simulink model "FOC"  (R2021a)
settings: Solver=VariableStepAuto  StartTime=0.0  StopTime=10  FixedStep=10e-5
InitFcn:
  | cd 'F:\Learning\Power\FOC';
  | run('Params.m')
values from neighbouring files (symbols this model uses):
  B = 1e-4    (= 0.0001)    [Params.m]
  Id_max = -62.5    [Params.m]
  Iq_max = 62.5    [Params.m]
  Is_max = 125    [Params.m]
  J = 0.004    [Params.m]
  Ka_id = 1 / Kp_id    (= 0.0111111111111)    [Params.m]
  Ka_iq = 1 / Kp_iq    (= 2.06143063286)    [Params.m]
  Ka_w = 1 / Kp_w    (= 0.1)    [Params.m]
  Kest = Rs/Ls    (= 212.401995723)    [Params.m]
  Ki_id = 50    [Params.m]
  Ki_iq = 93.62    [Params.m]
  Ki_w = 15    [Params.m]
  Kp_id = 90    [Params.m]
  Kp_iq = 0.4851    [Params.m]
  Kp_ll = 2500000    [Params.m]
  Kp_w = 10    [Params.m]
  Kw_Y = 7.98e-3    (= 0.00798)    [Params.m]
  Ld = 6.31e-5    (= 6.31e-05)    [Params.m]
  Lq = 7.72e-5    (= 7.72e-05)    [Params.m]
  Ls = 7.015e-5    (= 7.015e-05)    [Params.m]
  p = 6    [Params.m]
  Rs = 0.0149    [Params.m]
  Te_max = 2.4    [Params.m]
  Te_min = -2.4    [Params.m]
  TL = 1.67    [Params.m]
  Ts = 1/fs    (= 5e-05)    [Params.m]
  Vs_max = V_DC / sqrt(3)    [Params.m]
  Ypm = 7.89e-3    (= 0.00789)    [Params.m]
undefined symbols (not defined in the file or in its folder): magnitude
libraries: spsMosfetLib x6, spsVoltageMeasurementLib x3, spsDCVoltageSourceLib x2, spsGroundLib x1, spspowerguiLib x1
settings Model: SimulationMode=rapid-accelerator  Creator=DEEL  LastModifiedBy=DEEL
settings SolverCC: ZeroCrossControl=DisableAll
settings OptimizationCC: DefaultParameterBehavior=Inlined  EnhancedBackFolding=on  PassReuseOutputArgsAs=Individual arguments  ZeroExternalMemoryAtStartup=off  ZeroInternalMemoryAtStartup=off  OptimizeBlockOrder=speed  DifferentSizesBufferReuse=on  OptimizationCustomize=off  EfficientTunableParamExpr=on
settings DebuggingCC: ParameterTunabilityLossMsg=error
settings SFSimCC: MATLABDynamicMemAlloc=off
settings RTWCC: SystemTargetFile=ert.tlc  TemplateMakefile=ert_default_tmf
settings CodeAppCC: ForceParamTrailComments=on  IgnoreCustomStorageClasses=off  OperatorAnnotations=on  SimulinkDataObjDesc=on  SFDataObjDesc=on  InsertBlockDesc=on
settings ERTTargetCC: TargetLangStandard=C99 (ISO)  GenerateSampleERTMain=on  InlinedParameterPlacement=NonHierarchical  RTWCAPISignals=on  RTWCAPIParams=on  ERTCustomFileTemplate=example_file_process.tlc

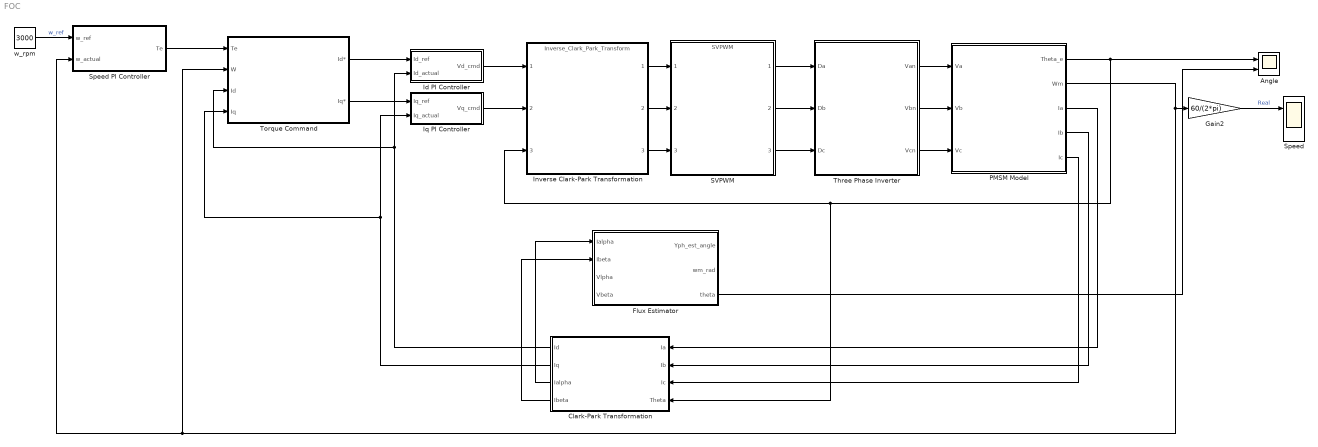
== system FOC ==
  Angle : Scope  NumInputPorts=2
  Clark-Park Transformation : Subsystem
  Flux Estimator : Subsystem
  Gain2 : Gain  Gain=60/(2*pi)
  Id PI Controller : Subsystem
  Inverse Clark-Park Transformation : ModelReference  ModelNameDialog=Inverse_Clark_Park_Transform  SimulationMode=Normal  ModelReferenceVersion=1.215
  Iq PI Controller : Subsystem
  PMSM Model : Subsystem
  SVPWM : ModelReference  ModelNameDialog=SVPWM  SimulationMode=Normal  ModelReferenceVersion=1.224
  Speed : Scope  NumInputPorts=2
  Speed PI Controller : Subsystem
  Three Phase Inverter : Subsystem
  Torque Command : Subsystem
  w_rpm : Constant  Value=3000
  wires:
  w_rpm/1 -> Speed PI Controller/1(w_ref)  "w_ref"
  Speed PI Controller/1(Te) -> Torque Command/1(Te)
  Id PI Controller/1(Vd_cmd) -> Inverse Clark-Park Transformation/1
  Iq PI Controller/1(Vq_cmd) -> Inverse Clark-Park Transformation/2
  Torque Command/1(Id*) -> Id PI Controller/1(Id_ref)
  SVPWM/3 -> Three Phase Inverter/3(Dc)
  SVPWM/1 -> Three Phase Inverter/1(Da)
  Inverse Clark-Park Transformation/1 -> SVPWM/1
  Inverse Clark-Park Transformation/2 -> SVPWM/2
  Inverse Clark-Park Transformation/3 -> SVPWM/3
  Clark-Park Transformation/1(Id) -> Torque Command/3(Id), Id PI Controller/2(Id_actual)
  Three Phase Inverter/1(Van) -> PMSM Model/1(Va)
  Three Phase Inverter/3(Vcn) -> PMSM Model/3(Vc)
  PMSM Model/3(Ia) -> Clark-Park Transformation/1(Ia)
  PMSM Model/4(Ib) -> Clark-Park Transformation/2(Ib)
  PMSM Model/5(Ic) -> Clark-Park Transformation/3(Ic)
  PMSM Model/2(Wm) -> Torque Command/2(W), Speed PI Controller/2(w_actual), Gain2/1
  PMSM Model/1(Theta_e) -> Clark-Park Transformation/4(Theta), Inverse Clark-Park Transformation/3, Angle/1
  Clark-Park Transformation/2(Iq) -> Torque Command/4(Iq), Iq PI Controller/2(Iq_actual)
  Three Phase Inverter/2(Vbn) -> PMSM Model/2(Vb)
  SVPWM/2 -> Three Phase Inverter/2(Db)
  Gain2/1 -> Speed/1  "Real"
  Torque Command/2(Iq*) -> Iq PI Controller/1(Iq_ref)
  Clark-Park Transformation/3(Ialpha) -> Flux Estimator/1(Ialpha)
  Clark-Park Transformation/4(Ibeta) -> Flux Estimator/2(Ibeta)
  Flux Estimator/3(theta) -> Angle/2

== system FOC/Clark-Park Transformation ==
  Ia : Inport
  Ib : Inport  Port=2
  Ic : Inport  Port=3
  Theta : Inport  Port=4
  Clark Transformation : Subsystem
  Park Transformation : Subsystem
  Id : Outport
  Iq : Outport  Port=2
  Ialpha : Outport  Port=3
  Ibeta : Outport  Port=4
  wires:
  Theta/1 -> Park Transformation/3(Theta)
  Clark Transformation/2(Vbeta) -> Ibeta/1, Park Transformation/2(Vbeta)
  Clark Transformation/1(Valpha) -> Ialpha/1, Park Transformation/1(Valpha)
  Ic/1 -> Clark Transformation/3(Vc)
  Ib/1 -> Clark Transformation/2(Vb)
  Ia/1 -> Clark Transformation/1(Va)
  Park Transformation/2(Vq) -> Iq/1
  Park Transformation/1(Vd) -> Id/1

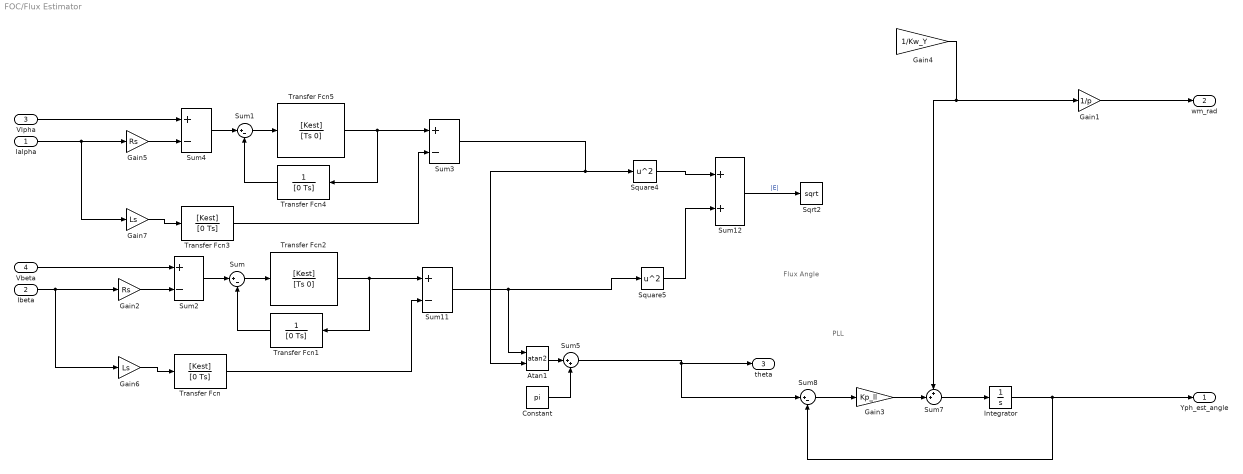
== system FOC/Flux Estimator ==
  note: PLL
  note: Flux Angle
  Ialpha : Inport
  Ibeta : Inport  Port=2
  Vlpha : Inport  Port=3
  Vbeta : Inport  Port=4
  Atan1 : Trigonometry  Operator=atan2
  Constant : Constant  Value=pi
  Gain1 : Gain  Gain=1/p
  Gain2 : Gain  Gain=Rs
  Gain3 : Gain  Gain=Kp_ll
  Gain4 : Gain  Gain=1/Kw_Y
  Gain5 : Gain  Gain=Rs
  Gain6 : Gain  Gain=Ls
  Gain7 : Gain  Gain=Ls
  Integrator : Integrator
  Sqrt2 : Sqrt  SaturateOnIntegerOverflow=on
  Square4 : Math  Operator=square  SaturateOnIntegerOverflow=on
  Square5 : Math  Operator=square  SaturateOnIntegerOverflow=on
  Sum : Sum  Inputs=|+-
  Sum1 : Sum  Inputs=|+-
  Sum{2..4,11} (4 alike) : Sum  Inputs=+-
  Sum12 : Sum
  Sum5 : Sum  Inputs=|++
  Sum7 : Sum  Inputs=++|
  Sum8 : Sum  Inputs=|+-
  Transfer Fcn : TransferFcn  Numerator=[Kest]  Denominator=[0 Ts]
  Transfer Fcn1 : TransferFcn  Denominator=[0 Ts]
  Transfer Fcn2 : TransferFcn  Numerator=[Kest]  Denominator=[Ts 0]
  Transfer Fcn3 : TransferFcn  Numerator=[Kest]  Denominator=[0 Ts]
  Transfer Fcn4 : TransferFcn  Denominator=[0 Ts]
  Transfer Fcn5 : TransferFcn  Numerator=[Kest]  Denominator=[Ts 0]
  Yph_est_angle : Outport
  wm_rad : Outport  Port=2
  theta : Outport  Port=3
  wires:
  Gain2/1 -> Sum2/2
  Ibeta/1 -> Gain6/1, Gain2/1
  Gain1/1 -> wm_rad/1
  Sum7/1 -> Integrator/1
  Sum8/1 -> Gain3/1
  Vbeta/1 -> Sum2/1
  Gain4/1 -> Sum7/1, Gain1/1
  Integrator/1 -> Yph_est_angle/1, Sum8/2
  Gain3/1 -> Sum7/2
  Square5/1 -> Sum12/2
  Square4/1 -> Sum12/1
  Sum12/1 -> Sqrt2/1  "|E|"
  Sum3/1 -> Atan1/2, Square4/1
  Sum11/1 -> Square5/1, Atan1/1
  Sum5/1 -> Sum8/1, theta/1
  Gain6/1 -> Transfer Fcn/1
  Sum/1 -> Transfer Fcn2/1
  Sum2/1 -> Sum/1
  Transfer Fcn1/1 -> Sum/2
  Transfer Fcn2/1 -> Transfer Fcn1/1, Sum11/1
  Transfer Fcn/1 -> Sum11/2
  Transfer Fcn3/1 -> Sum3/2
  Transfer Fcn5/1 -> Sum3/1, Transfer Fcn4/1
  Transfer Fcn4/1 -> Sum1/2
  Sum4/1 -> Sum1/1
  Sum1/1 -> Transfer Fcn5/1
  Gain7/1 -> Transfer Fcn3/1
  Vlpha/1 -> Sum4/1
  Ialpha/1 -> Gain7/1, Gain5/1
  Gain5/1 -> Sum4/2
  Atan1/1 -> Sum5/1
  Constant/1 -> Sum5/2

== system FOC/Id PI Controller ==
  Id_ref : Inport
  Id_actual : Inport  Port=2
  Gain : Gain  Gain=Kp_id
  Gain1 : Gain  Gain=Ki_id
  Gain2 : Gain  Gain=Ka_id
  Integrator : Integrator
  Saturation : Saturate  UpperLimit=Vs_max  LowerLimit=-Vs_max
  Sum : Sum  Inputs=|+-
  Sum1 : Sum  Inputs=|++
  Sum2 : Sum  Inputs=+-|
  Sum3 : Sum  Inputs=|+-
  Vd_cmd : Outport
  wires:
  Sum1/1 -> Sum2/1, Saturation/1  "Voltage_Command"
  Integrator/1 -> Sum1/2
  Gain/1 -> Sum1/1
  Gain1/1 -> Integrator/1
  Sum/1 -> Sum3/1, Gain/1  "Id_err"
  Id_actual/1 -> Sum/2
  Id_ref/1 -> Sum/1
  Sum2/1 -> Gain2/1
  Gain2/1 -> Sum3/2  "Anti-WindUp"
  Saturation/1 -> Sum2/2, Vd_cmd/1
  Sum3/1 -> Gain1/1  "Id_err"

== system FOC/Iq PI Controller ==
  Iq_ref : Inport
  Iq_actual : Inport  Port=2
  Gain : Gain  Gain=Kp_iq
  Gain1 : Gain  Gain=Ki_iq
  Gain2 : Gain  Gain=Ka_iq
  Integrator : Integrator
  Saturation1 : Saturate  UpperLimit=Vs_max  LowerLimit=-Vs_max
  Sum : Sum  Inputs=|+-
  Sum1 : Sum  Inputs=|++
  Sum2 : Sum  Inputs=+-|
  Sum3 : Sum  Inputs=|+-
  Vq_cmd : Outport
  wires:
  Gain1/1 -> Integrator/1
  Gain/1 -> Sum1/1
  Integrator/1 -> Sum1/2
  Sum1/1 -> Sum2/1, Saturation1/1  "Voltage_Command"
  Iq_actual/1 -> Sum/2
  Iq_ref/1 -> Sum/1
  Sum2/1 -> Gain2/1
  Saturation1/1 -> Sum2/2, Vq_cmd/1
  Gain2/1 -> Sum3/2  "Anti-WindUp"
  Sum/1 -> Sum3/1, Gain/1  "Iq_err"
  Sum3/1 -> Gain1/1  "Iq_err"

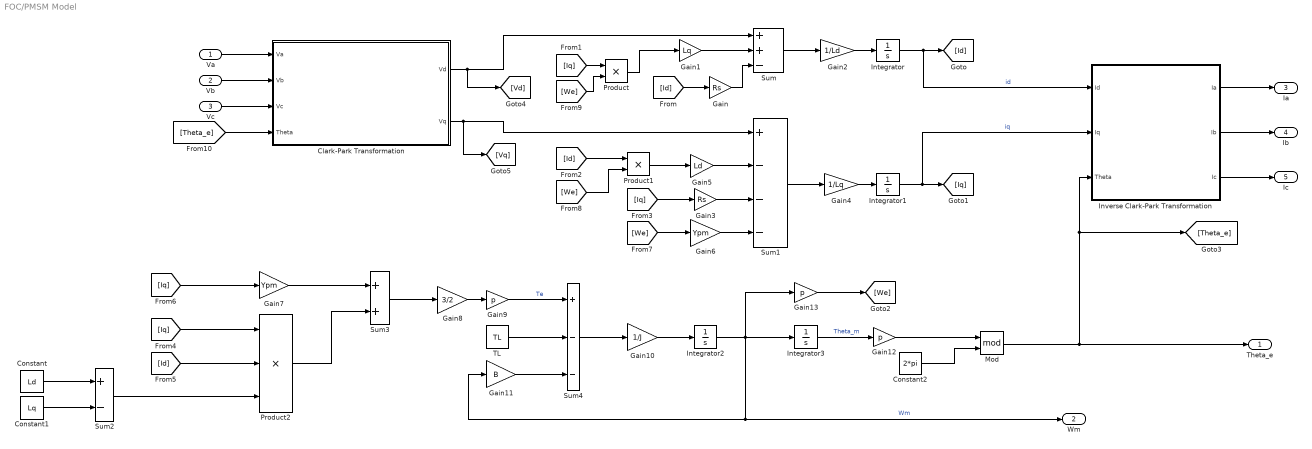
== system FOC/PMSM Model ==
  Va : Inport
  Vb : Inport  Port=2
  Vc : Inport  Port=3
  Clark-Park Transformation : Subsystem
  Constant : Constant  Value=Ld
  Constant1 : Constant  Value=Lq
  Constant2 : Constant  Value=2*pi
  Gain : Gain  Gain=Rs
  Gain1 : Gain  Gain=Lq
  Gain10 : Gain  Gain=1/J
  Gain11 : Gain  Gain=B
  Gain12 : Gain  Gain=p
  Gain13 : Gain  Gain=p
  Gain2 : Gain  Gain=1/Ld
  Gain3 : Gain  Gain=Rs
  Gain4 : Gain  Gain=1/Lq
  Gain5 : Gain  Gain=Ld
  Gain6 : Gain  Gain=Ypm
  Gain7 : Gain  Gain=Ypm
  Gain8 : Gain  Gain=3/2
  Gain9 : Gain  Gain=p
  Integrator{,1..3} (4 alike) : Integrator
  Inverse Clark-Park Transformation : Subsystem
  Mod : Math  Operator=mod  SaturateOnIntegerOverflow=on
  Product : Product
  Product1 : Product
  Product2 : Product  Inputs=3
  Sum : Sum  Inputs=++-
  Sum1 : Sum  Inputs=+---
  Sum2 : Sum  Inputs=+-
  Sum3 : Sum
  Sum4 : Sum  Inputs=+--
  TL : Constant  Value=TL
  Theta_e : Outport
  Wm : Outport  Port=2
  Ia : Outport  Port=3
  Ib : Outport  Port=4
  Ic : Outport  Port=5
  wires:
  Vc/1 -> Clark-Park Transformation/3(Vc)
  Va/1 -> Clark-Park Transformation/1(Va)
  Clark-Park Transformation/1(Vd) -> [Vd], Sum/1
  Gain/1 -> Sum/3
  Product/1 -> Gain1/1
  Sum/1 -> Gain2/1
  Gain2/1 -> Integrator/1
  Gain1/1 -> Sum/2
  Clark-Park Transformation/2(Vq) -> [Vq], Sum1/1
  Sum1/1 -> Gain4/1
  Gain4/1 -> Integrator1/1
  Gain3/1 -> Sum1/3
  Product1/1 -> Gain5/1
  Gain5/1 -> Sum1/2
  Integrator/1 -> Inverse Clark-Park Transformation/1(Id), [Id]  "id"
  [Id] -> Gain/1
  Integrator1/1 -> Inverse Clark-Park Transformation/2(Iq), [Iq]  "iq"
  [Iq] -> Product/1
  [Id] -> Product1/1
  [Iq] -> Gain3/1
  Gain6/1 -> Sum1/4
  [Iq] -> Product2/1
  [Id] -> Product2/2
  Sum2/1 -> Product2/3
  Constant1/1 -> Sum2/2
  Constant/1 -> Sum2/1
  [Iq] -> Gain7/1
  Gain7/1 -> Sum3/1
  Product2/1 -> Sum3/2
  Sum3/1 -> Gain8/1
  Sum4/1 -> Gain10/1
  TL/1 -> Sum4/2
  Gain11/1 -> Sum4/3
  Gain10/1 -> Integrator2/1
  Integrator2/1 -> Gain13/1, Integrator3/1, Wm/1, Gain11/1  "Wm"
  Integrator3/1 -> Gain12/1  "Theta_m"
  Gain13/1 -> [We]
  [We] -> Gain6/1
  [We] -> Product1/2
  [We] -> Product/2
  Gain12/1 -> Mod/1
  Constant2/1 -> Mod/2
  [Theta_e] -> Clark-Park Transformation/4(Theta)
  Gain8/1 -> Gain9/1
  Gain9/1 -> Sum4/1  "Te"
  Mod/1 -> Theta_e/1, Inverse Clark-Park Transformation/3(Theta), [Theta_e]
  Vb/1 -> Clark-Park Transformation/2(Vb)
  Inverse Clark-Park Transformation/1(Ia) -> Ia/1
  Inverse Clark-Park Transformation/2(Ib) -> Ib/1
  Inverse Clark-Park Transformation/3(Ic) -> Ic/1

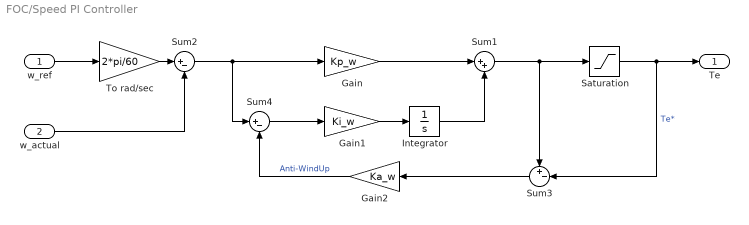
== system FOC/Speed PI Controller ==
  w_ref : Inport
  w_actual : Inport  Port=2
  Gain : Gain  Gain=Kp_w
  Gain1 : Gain  Gain=Ki_w
  Gain2 : Gain  Gain=Ka_w
  Integrator : Integrator
  Saturation : Saturate  UpperLimit=Te_max  LowerLimit=Te_min
  Sum1 : Sum  Inputs=|++
  Sum2 : Sum  Inputs=|+-
  Sum3 : Sum  Inputs=+-|
  Sum4 : Sum  Inputs=|+-
  To rad/sec : Gain  Gain=2*pi/60
  Te : Outport
  wires:
  Sum2/1 -> Sum4/1, Gain/1
  Integrator/1 -> Sum1/2
  Gain1/1 -> Integrator/1
  Saturation/1 -> Sum3/2, Te/1  "Te*"
  w_ref/1 -> To rad/sec/1
  Sum3/1 -> Gain2/1
  Sum1/1 -> Saturation/1, Sum3/1
  Gain2/1 -> Sum4/2  "Anti-WindUp"
  Sum4/1 -> Gain1/1
  To rad/sec/1 -> Sum2/1
  Gain/1 -> Sum1/1
  w_actual/1 -> Sum2/2

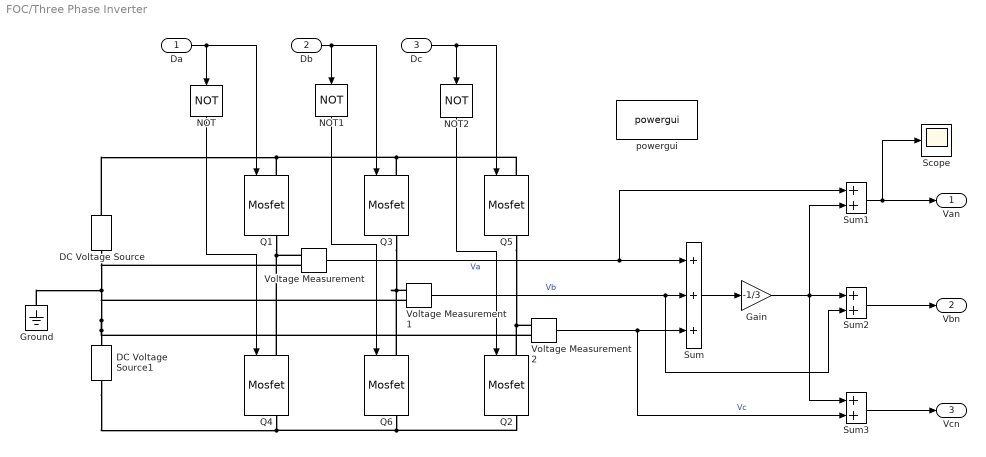
== system FOC/Three Phase Inverter ==
  Da : Inport  OutDataTypeStr=boolean  PortDimensions=1  SampleTime=[4.9999999999999998e-07,0]
  Db : Inport  Port=2  OutDataTypeStr=boolean  PortDimensions=1  SampleTime=[4.9999999999999998e-07,0]
  Dc : Inport  Port=3  OutDataTypeStr=boolean  PortDimensions=1  SampleTime=[4.9999999999999998e-07,0]
  DC Voltage Source : spsDCVoltageSourceLib/DC Voltage Source  Amplitude=12  Measurements=None
  DC Voltage Source1 : spsDCVoltageSourceLib/DC Voltage Source  Amplitude=12  Measurements=None
  Gain : Gain  Gain=-1/3
  Ground : spsGroundLib/Ground  LConnTagsString=a
  NOT : Logic  Operator=NOT  IconShape=distinctive  AllPortsSameDT=off  OutDataTypeStr=boolean
  NOT1 : Logic  Operator=NOT  IconShape=distinctive  AllPortsSameDT=off  OutDataTypeStr=boolean
  NOT2 : Logic  Operator=NOT  IconShape=distinctive  AllPortsSameDT=off  OutDataTypeStr=boolean
  Q{1..6} (6 alike) : spsMosfetLib/Mosfet  Ron=0.1  Lon=0  Rd=0.01  Vfd=0  IC=0  Rs=1e5  Cs=inf  Measurements=on
  Scope : Scope
  Sum : Sum  Inputs=+++
  Sum1 : Sum
  Sum2 : Sum
  Sum3 : Sum
  Voltage Measurement : spsVoltageMeasurementLib/Voltage Measurement  PhasorSimulation=off  OutputType=Complex  PSBequivalent=0
  Voltage Measurement1 : spsVoltageMeasurementLib/Voltage Measurement  PhasorSimulation=off  OutputType=Complex  PSBequivalent=0
  Voltage Measurement2 : spsVoltageMeasurementLib/Voltage Measurement  PhasorSimulation=off  OutputType=Complex  PSBequivalent=0
  powergui : spspowerguiLib/powergui  Priority=1  SimulationMode=Continuous  SampleTime=50e-6  frequency=60  Iterations=50  frequencyindice=0  Pbase=100e6  ErrMax=1e-4  UnitsV=kV  UnitsW=MW  buscounter=0  FunctionMessages=off  echomessages=off  EnableUseOfTLC=off  CurrentSourceSwitches=off  DisableSnubberDevices=off  DisableRonSwitches=off  DisableVfSwitches=off  DisplayEquations=off  AutomaticDiscreteSolvers=off  SolverType=Tustin/Backward Euler (TBE)  Interpol=off  ExternalGateDelay=off  methode=off  Ts=100  x0status=blocks  SPID=on  SwTol=0  HookPort=off  NonlinearTolerance=1e-4  nMaxIteration=100  ContinueOnMaxIteration=off  RestoreLinks=warning  ResistiveCurrentMeasurement=off  Frange=[0:2:500]  Ylog=off  Xlog=on  ShowGrid=off  save=off  variable=ZData  structure=0  ZoomFFT=off  StartTime=0.0  cycles=1  DisplayStyle=1  fundamental=60  FreqAxis=off  MaxFrequency=1000  frequencyindicesteady=1  RmsSteady=1  display=off
  Van : Outport  OutDataTypeStr=double  PortDimensions=1  SampleTime=0
  Vbn : Outport  Port=2  OutDataTypeStr=double  PortDimensions=1  SampleTime=0
  Vcn : Outport  Port=3  OutDataTypeStr=double  PortDimensions=1  SampleTime=0
  wires:
  NOT2/1 -> Q2/1
  NOT1/1 -> Q6/1
  Db/1 -> NOT1/1, Q3/1
  Da/1 -> NOT/1, Q1/1
  NOT/1 -> Q4/1
  Dc/1 -> NOT2/1, Q5/1
  Voltage Measurement/1 -> Sum1/1, Sum/1  "Va"
  Voltage Measurement1/1 -> Sum2/2, Sum/2  "Vb"
  Voltage Measurement2/1 -> Sum3/2, Sum/3  "Vc"
  Sum/1 -> Gain/1
  Sum1/1 -> Scope/1, Van/1
  Gain/1 -> Sum3/1, Sum2/1, Sum1/2
  Sum2/1 -> Vbn/1
  Sum3/1 -> Vcn/1
  connections:
  Voltage Measurement/LConn1 -- Q4/LConn1 -- Q1/RConn1
  Q2/RConn1 -- DC Voltage Source1/LConn1 -- Q4/RConn1 -- Q6/RConn1
  Voltage Measurement1/LConn1 -- Q3/RConn1 -- Q6/LConn1
  Q3/LConn1 -- Q5/LConn1 -- DC Voltage Source/RConn1 -- Q1/LConn1
  Voltage Measurement2/LConn2 -- DC Voltage Source/LConn1 -- Voltage Measurement/LConn2 -- Ground/LConn1 -- Voltage Measurement1/LConn2 -- DC Voltage Source1/RConn1
  Voltage Measurement2/LConn1 -- Q5/RConn1 -- Q2/LConn1

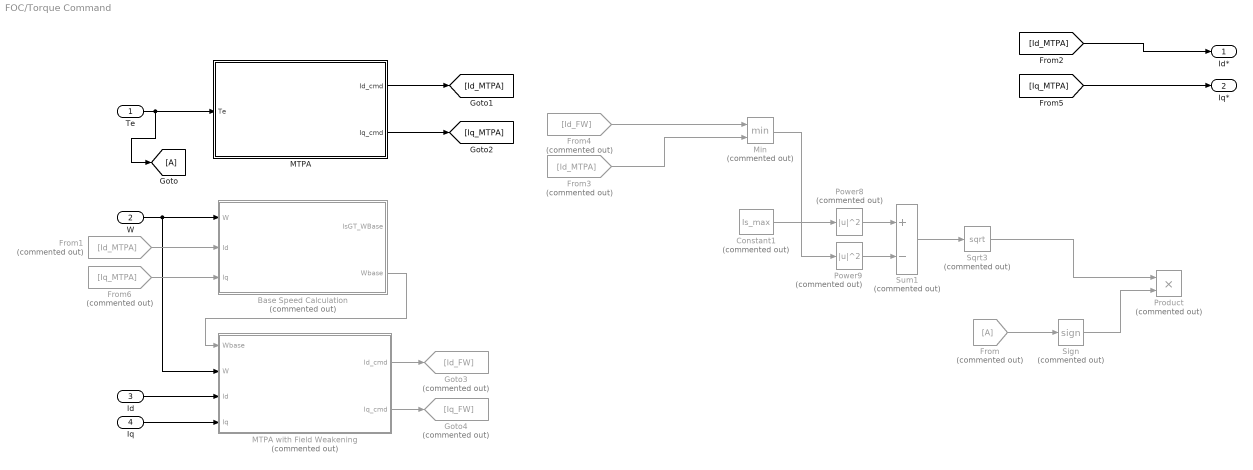
== system FOC/Torque Command ==
  Te : Inport
  W : Inport  Port=2
  Id : Inport  Port=3
  Iq : Inport  Port=4
  Base Speed Calculation : Subsystem  Commented=on
  Constant1 : Constant  Commented=on  Value=Is_max
  From : From  Commented=on
  From1 : From  Commented=on  GotoTag=Id_MTPA
  From3 : From  Commented=on  GotoTag=Id_MTPA
  From4 : From  Commented=on  GotoTag=Id_FW
  From6 : From  Commented=on  GotoTag=Iq_MTPA
  Goto3 : Goto  Commented=on  GotoTag=Id_FW
  Goto4 : Goto  Commented=on  GotoTag=Iq_FW
  MTPA : Subsystem
  MTPA with Field Weakening : Subsystem  Commented=on
  Min : MinMax  Commented=on  Inputs=2
  Power8 : Math  Commented=on  Operator=magnitude^2  SaturateOnIntegerOverflow=on
  Power9 : Math  Commented=on  Operator=magnitude^2  SaturateOnIntegerOverflow=on
  Product : Product  Commented=on
  Sign : Signum  Commented=on
  Sqrt3 : Sqrt  Commented=on  SaturateOnIntegerOverflow=on
  Sum1 : Sum  Commented=on  Inputs=+-
  Id* : Outport
  Iq* : Outport  Port=2
  wires:
  W/1 -> MTPA with Field Weakening/2(W), Base Speed Calculation/1(W)
  MTPA/2(Iq_cmd) -> [Iq_MTPA]
  MTPA/1(Id_cmd) -> [Id_MTPA]
  MTPA with Field Weakening/1(Id_cmd) -> Goto3/1
  MTPA with Field Weakening/2(Iq_cmd) -> Goto4/1
  Base Speed Calculation/2(Wbase) -> MTPA with Field Weakening/1(Wbase)
  From1/1 -> Base Speed Calculation/2(Id)
  From6/1 -> Base Speed Calculation/3(Iq)
  From4/1 -> Min/1
  From3/1 -> Min/2
  Power8/1 -> Sum1/1
  Power9/1 -> Sum1/2
  Constant1/1 -> Power8/1
  Sum1/1 -> Sqrt3/1
  Min/1 -> Power9/1
  Te/1 -> [A], MTPA/1(Te)
  From/1 -> Sign/1
  Sign/1 -> Product/2
  Sqrt3/1 -> Product/1
  Id/1 -> MTPA with Field Weakening/3(Id)
  Iq/1 -> MTPA with Field Weakening/4(Iq)
  [Iq_MTPA] -> Iq*/1
  [Id_MTPA] -> Id*/1

== system FOC/Clark-Park Transformation/Clark Transformation ==
  Va : Inport
  Vb : Inport  Port=2
  Vc : Inport  Port=3
  Constant : Constant  Value=[1 ,-1/2,-1/2;0,sqrt(3)/2,-sqrt(3)/2]
  Demux : Demux  Outputs=2
  MatrixMultiply : Product  Multiplication=Matrix(*)
  Mux : Mux  Inputs=3
  Valpha : Outport
  Vbeta : Outport  Port=2
  wires:
  Va/1 -> Mux/1
  Vb/1 -> Mux/2
  Vc/1 -> Mux/3
  Constant/1 -> MatrixMultiply/1
  Mux/1 -> MatrixMultiply/2
  MatrixMultiply/1 -> Demux/1
  Demux/1 -> Valpha/1
  Demux/2 -> Vbeta/1

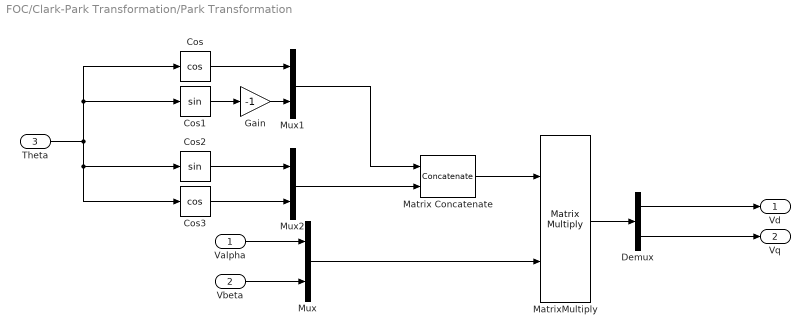
== system FOC/Clark-Park Transformation/Park Transformation ==
  Valpha : Inport
  Vbeta : Inport  Port=2
  Theta : Inport  Port=3
  Cos : Trigonometry  Operator=cos
  Cos1 : Trigonometry
  Cos2 : Trigonometry
  Cos3 : Trigonometry  Operator=cos
  Demux : Demux  Outputs=2
  Gain : Gain  Gain=-1
  Matrix Concatenate : Concatenate  Mode=Multidimensional array  ConcatenateDimension=2
  MatrixMultiply : Product  Multiplication=Matrix(*)
  Mux : Mux  Inputs=2
  Mux1 : Mux  Inputs=2
  Mux2 : Mux  Inputs=2
  Vd : Outport
  Vq : Outport  Port=2
  wires:
  Demux/2 -> Vq/1
  Demux/1 -> Vd/1
  MatrixMultiply/1 -> Demux/1
  Mux/1 -> MatrixMultiply/2
  Valpha/1 -> Mux/1
  Cos3/1 -> Mux2/2
  Gain/1 -> Mux1/2
  Mux2/1 -> Matrix Concatenate/2
  Cos/1 -> Mux1/1
  Mux1/1 -> Matrix Concatenate/1
  Theta/1 -> Cos/1, Cos1/1, Cos3/1, Cos2/1
  Cos1/1 -> Gain/1
  Cos2/1 -> Mux2/1
  Vbeta/1 -> Mux/2
  Matrix Concatenate/1 -> MatrixMultiply/1

== system FOC/PMSM Model/Clark-Park Transformation ==
  Va : Inport
  Vb : Inport  Port=2
  Vc : Inport  Port=3
  Theta : Inport  Port=4
  Clark Transformation : Subsystem
  Park Transformation : Subsystem
  Vd : Outport
  Vq : Outport  Port=2
  wires:
  Clark Transformation/1(Valpha) -> Park Transformation/1(Valpha)
  Vc/1 -> Clark Transformation/3(Vc)
  Vb/1 -> Clark Transformation/2(Vb)
  Va/1 -> Clark Transformation/1(Va)
  Park Transformation/1(Vd) -> Vd/1
  Park Transformation/2(Vq) -> Vq/1
  Clark Transformation/2(Vbeta) -> Park Transformation/2(Vbeta)
  Theta/1 -> Park Transformation/3(Theta)

== system FOC/PMSM Model/Inverse Clark-Park Transformation ==
  Id : Inport
  Iq : Inport  Port=2
  Theta : Inport  Port=3
  Gain : Gain  Gain=2/3
  Gain1 : Gain  Gain=2/3
  Gain2 : Gain  Gain=2/3
  Inverse-Clark Transformation : Subsystem
  Inverse-Park Transformation : Subsystem
  Ia : Outport
  Ib : Outport  Port=2
  Ic : Outport  Port=3
  wires:
  Inverse-Clark Transformation/2(Vb) -> Gain1/1
  Inverse-Clark Transformation/1(Va) -> Gain/1
  Inverse-Park Transformation/2(Vbeta) -> Inverse-Clark Transformation/2(Vbeta)
  Inverse-Park Transformation/1(Valpha) -> Inverse-Clark Transformation/1(Valpha)
  Inverse-Clark Transformation/3(Vc) -> Gain2/1
  Iq/1 -> Inverse-Park Transformation/2(Vq)
  Id/1 -> Inverse-Park Transformation/1(Vd)
  Theta/1 -> Inverse-Park Transformation/3(Theta)
  Gain/1 -> Ia/1
  Gain1/1 -> Ib/1
  Gain2/1 -> Ic/1

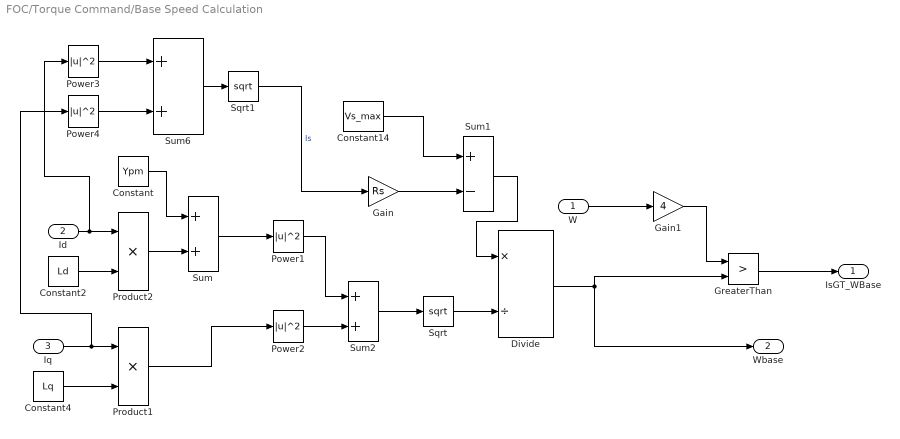
== system FOC/Torque Command/Base Speed Calculation ==
  W : Inport
  Id : Inport  Port=2
  Iq : Inport  Port=3
  Constant : Constant  Value=Ypm
  Constant14 : Constant  Value=Vs_max
  Constant2 : Constant  Value=Ld
  Constant4 : Constant  Value=Lq
  Divide : Product  Inputs=*/
  Gain : Gain  Gain=Rs
  Gain1 : Gain  Gain=4
  GreaterThan : RelationalOperator  Operator=>  OutDataTypeStr=boolean  RndMeth=Simplest
  Power{1..4} (4 alike) : Math  Operator=magnitude^2  SaturateOnIntegerOverflow=on
  Product1 : Product
  Product2 : Product
  Sqrt : Sqrt  SaturateOnIntegerOverflow=on
  Sqrt1 : Sqrt  SaturateOnIntegerOverflow=on
  Sum : Sum
  Sum1 : Sum  Inputs=+-
  Sum2 : Sum
  Sum6 : Sum
  IsGT_WBase : Outport
  Wbase : Outport  Port=2
  wires:
  Constant/1 -> Sum/1
  Constant2/1 -> Product2/2
  Constant4/1 -> Product1/2
  Iq/1 -> Power4/1, Product1/1
  Id/1 -> Power3/1, Product2/1
  Product2/1 -> Sum/2
  Sum/1 -> Power1/1
  Product1/1 -> Power2/1
  Power2/1 -> Sum2/2
  Power1/1 -> Sum2/1
  Sum2/1 -> Sqrt/1
  Sqrt/1 -> Divide/2
  W/1 -> Gain1/1
  Divide/1 -> Wbase/1, GreaterThan/2
  GreaterThan/1 -> IsGT_WBase/1
  Constant14/1 -> Sum1/1
  Sum6/1 -> Sqrt1/1
  Power3/1 -> Sum6/1
  Power4/1 -> Sum6/2
  Sqrt1/1 -> Gain/1  "Is"
  Gain/1 -> Sum1/2
  Sum1/1 -> Divide/1
  Gain1/1 -> GreaterThan/1

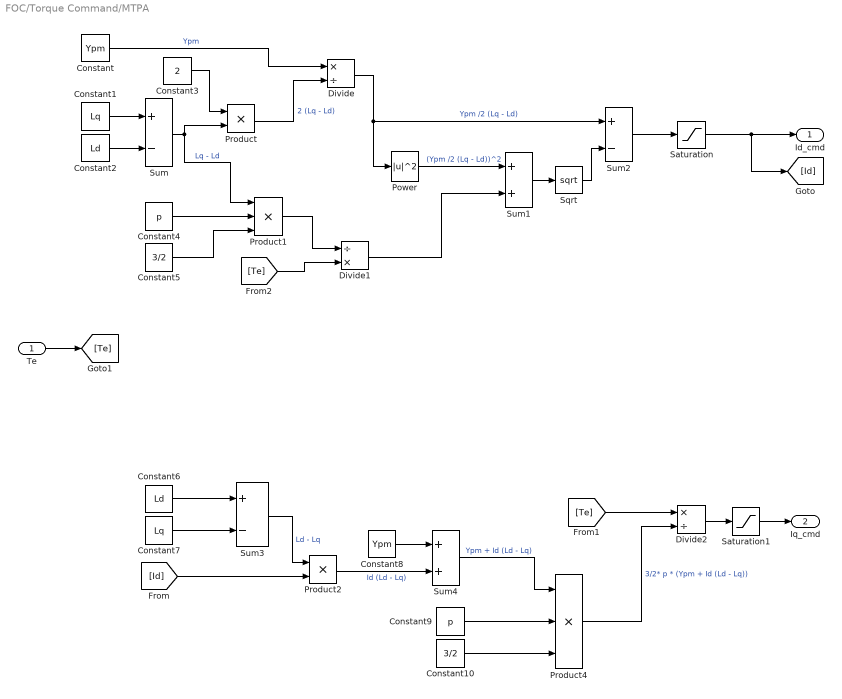
== system FOC/Torque Command/MTPA ==
  Te : Inport
  Constant : Constant  Value=Ypm
  Constant1 : Constant  Value=Lq
  Constant10 : Constant  Value=3/2
  Constant2 : Constant  Value=Ld
  Constant3 : Constant  Value=2
  Constant4 : Constant  Value=p
  Constant5 : Constant  Value=3/2
  Constant6 : Constant  Value=Ld
  Constant7 : Constant  Value=Lq
  Constant8 : Constant  Value=Ypm
  Constant9 : Constant  Value=p
  Divide : Product  Inputs=*/
  Divide1 : Product  Inputs=/*
  Divide2 : Product  Inputs=*/
  Power : Math  Operator=magnitude^2  SaturateOnIntegerOverflow=on
  Product : Product
  Product1 : Product  Inputs=3
  Product2 : Product
  Product4 : Product  Inputs=3
  Saturation : Saturate  UpperLimit=-Id_max  LowerLimit=Id_max
  Saturation1 : Saturate  UpperLimit=Iq_max  LowerLimit=-Iq_max
  Sqrt : Sqrt  SaturateOnIntegerOverflow=on
  Sum : Sum  Inputs=+-
  Sum1 : Sum
  Sum2 : Sum  Inputs=+-
  Sum3 : Sum  Inputs=+-
  Sum4 : Sum
  Id_cmd : Outport
  Iq_cmd : Outport  Port=2
  wires:
  [Te] -> Divide2/1
  [Te] -> Divide1/2
  Constant9/1 -> Product4/2
  Sqrt/1 -> Sum2/2
  Sum3/1 -> Product2/1  "Ld - Lq"
  Divide/1 -> Sum2/1, Power/1  "Ypm /2 (Lq - Ld)"
  [Id] -> Product2/2
  Product2/1 -> Sum4/2  "Id (Ld - Lq)"
  Constant10/1 -> Product4/3
  Constant8/1 -> Sum4/1
  Divide1/1 -> Sum1/2
  Sum4/1 -> Product4/1  "Ypm + Id (Ld - Lq)"
  Product4/1 -> Divide2/2  "3/2* p * (Ypm + Id (Ld - Lq))"
  Constant6/1 -> Sum3/1
  Sum/1 -> Product/2, Product1/1  "Lq - Ld"
  Power/1 -> Sum1/1  "(Ypm /2 (Lq - Ld))^2"
  Product/1 -> Divide/2  "2 (Lq - Ld)"
  Constant3/1 -> Product/1
  Constant4/1 -> Product1/2
  Sum1/1 -> Sqrt/1
  Constant1/1 -> Sum/1
  Product1/1 -> Divide1/1
  Constant5/1 -> Product1/3
  Constant7/1 -> Sum3/2
  Constant2/1 -> Sum/2
  Constant/1 -> Divide/1  "Ypm"
  Te/1 -> [Te]
  Divide2/1 -> Saturation1/1
  Sum2/1 -> Saturation/1
  Saturation/1 -> [Id], Id_cmd/1
  Saturation1/1 -> Iq_cmd/1

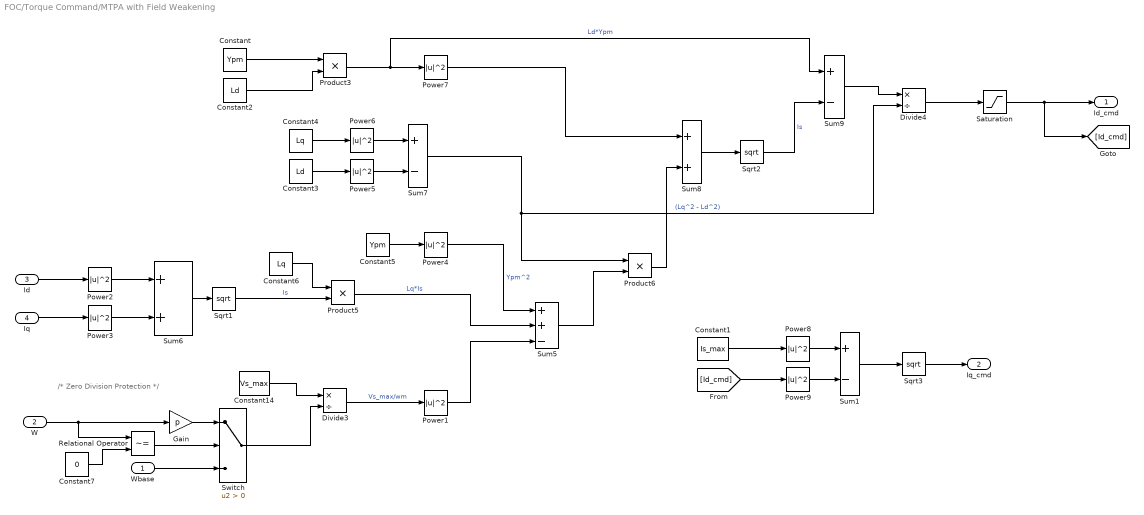
== system FOC/Torque Command/MTPA with Field Weakening ==
  note: /* Zero Division Protection */
  Wbase : Inport
  W : Inport  Port=2
  Id : Inport  Port=3
  Iq : Inport  Port=4
  Constant : Constant  Value=Ypm
  Constant1 : Constant  Value=Is_max
  Constant14 : Constant  Value=Vs_max
  Constant2 : Constant  Value=Ld
  Constant3 : Constant  Value=Ld
  Constant4 : Constant  Value=Lq
  Constant5 : Constant  Value=Ypm
  Constant6 : Constant  Value=Lq
  Constant7 : Constant  Value=0
  Divide3 : Product  Inputs=*/
  Divide4 : Product  Inputs=*/
  Gain : Gain  Gain=p
  Power{1..9} (9 alike) : Math  Operator=magnitude^2  SaturateOnIntegerOverflow=on
  Product3 : Product
  Product5 : Product
  Product6 : Product
  Relational Operator : RelationalOperator  Operator=~=  OutDataTypeStr=boolean  RndMeth=Simplest
  Saturation : Saturate  UpperLimit=Is_max  LowerLimit=-Is_max
  Sqrt1 : Sqrt  SaturateOnIntegerOverflow=on
  Sqrt2 : Sqrt  SaturateOnIntegerOverflow=on
  Sqrt3 : Sqrt  SaturateOnIntegerOverflow=on
  Sum1 : Sum  Inputs=+-
  Sum5 : Sum  Inputs=++-
  Sum6 : Sum
  Sum7 : Sum  Inputs=+-
  Sum8 : Sum
  Sum9 : Sum  Inputs=+-
  Switch : Switch  Criteria=u2 > Threshold
  Id_cmd : Outport
  Iq_cmd : Outport  Port=2
  wires:
  Product5/1 -> Sum5/2  "Lq*Is"
  Sum9/1 -> Divide4/1
  Sqrt1/1 -> Product5/2  "Is"
  Sqrt2/1 -> Sum9/2  "Is"
  Constant2/1 -> Product3/2
  Power5/1 -> Sum7/2
  Iq/1 -> Power3/1
  Product3/1 -> Sum9/1, Power7/1  "Ld*Ypm"
  Power7/1 -> Sum8/1
  Constant14/1 -> Divide3/1
  Power1/1 -> Sum5/3
  Id/1 -> Power2/1
  W/1 -> Relational Operator/1, Gain/1
  Divide4/1 -> Saturation/1
  Divide3/1 -> Power1/1  "Vs_max/wm"
  Power6/1 -> Sum7/1
  Product6/1 -> Sum8/2
  Constant4/1 -> Power6/1
  Power4/1 -> Sum5/1  "Ypm^2"
  Sum5/1 -> Product6/2
  Power3/1 -> Sum6/2
  Constant3/1 -> Power5/1
  Sum7/1 -> Divide4/2, Product6/1  "(Lq^2 - Ld^2)"
  Sum8/1 -> Sqrt2/1
  Power2/1 -> Sum6/1
  Sum6/1 -> Sqrt1/1
  Constant1/1 -> Power8/1
  Power8/1 -> Sum1/1
  Power9/1 -> Sum1/2
  Sum1/1 -> Sqrt3/1
  Sqrt3/1 -> Iq_cmd/1
  Constant/1 -> Product3/1
  Constant5/1 -> Power4/1
  Constant6/1 -> Product5/1
  [Id_cmd] -> Power9/1
  Relational Operator/1 -> Switch/2
  Switch/1 -> Divide3/2
  Constant7/1 -> Relational Operator/2
  Wbase/1 -> Switch/3
  Saturation/1 -> [Id_cmd], Id_cmd/1
  Gain/1 -> Switch/1

== system FOC/PMSM Model/Clark-Park Transformation/Clark Transformation ==
  Va : Inport
  Vb : Inport  Port=2
  Vc : Inport  Port=3
  Constant : Constant  Value=[1 ,-1/2,-1/2;0,sqrt(3)/2,-sqrt(3)/2]
  Demux : Demux  Outputs=2
  MatrixMultiply : Product  Multiplication=Matrix(*)
  Mux : Mux  Inputs=3
  Valpha : Outport
  Vbeta : Outport  Port=2
  wires:
  Va/1 -> Mux/1
  Vb/1 -> Mux/2
  Vc/1 -> Mux/3
  Constant/1 -> MatrixMultiply/1
  Mux/1 -> MatrixMultiply/2
  MatrixMultiply/1 -> Demux/1
  Demux/1 -> Valpha/1
  Demux/2 -> Vbeta/1

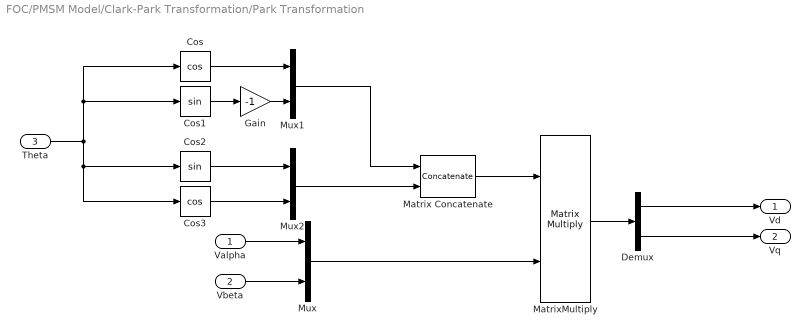
== system FOC/PMSM Model/Clark-Park Transformation/Park Transformation ==
  Valpha : Inport
  Vbeta : Inport  Port=2
  Theta : Inport  Port=3
  Cos : Trigonometry  Operator=cos
  Cos1 : Trigonometry
  Cos2 : Trigonometry
  Cos3 : Trigonometry  Operator=cos
  Demux : Demux  Outputs=2
  Gain : Gain  Gain=-1
  Matrix Concatenate : Concatenate  Mode=Multidimensional array  ConcatenateDimension=2
  MatrixMultiply : Product  Multiplication=Matrix(*)
  Mux : Mux  Inputs=2
  Mux1 : Mux  Inputs=2
  Mux2 : Mux  Inputs=2
  Vd : Outport
  Vq : Outport  Port=2
  wires:
  Demux/2 -> Vq/1
  Demux/1 -> Vd/1
  MatrixMultiply/1 -> Demux/1
  Mux/1 -> MatrixMultiply/2
  Valpha/1 -> Mux/1
  Cos3/1 -> Mux2/2
  Gain/1 -> Mux1/2
  Mux2/1 -> Matrix Concatenate/2
  Cos/1 -> Mux1/1
  Mux1/1 -> Matrix Concatenate/1
  Theta/1 -> Cos/1, Cos1/1, Cos3/1, Cos2/1
  Cos1/1 -> Gain/1
  Cos2/1 -> Mux2/1
  Vbeta/1 -> Mux/2
  Matrix Concatenate/1 -> MatrixMultiply/1

== system FOC/PMSM Model/Inverse Clark-Park Transformation/Inverse-Clark Transformation ==
  Valpha : Inport
  Vbeta : Inport  Port=2
  Constant : Constant  Value=[1 ,0;-1/2,sqrt(3)/2;-1/2,-sqrt(3)/2]
  Demux : Demux  Outputs=3
  MatrixMultiply : Product  Multiplication=Matrix(*)
  Mux : Mux  Inputs=2
  Va : Outport
  Vb : Outport  Port=2
  Vc : Outport  Port=3
  wires:
  Demux/2 -> Vb/1
  Demux/1 -> Va/1
  MatrixMultiply/1 -> Demux/1
  Mux/1 -> MatrixMultiply/2
  Constant/1 -> MatrixMultiply/1
  Vbeta/1 -> Mux/2
  Valpha/1 -> Mux/1
  Demux/3 -> Vc/1

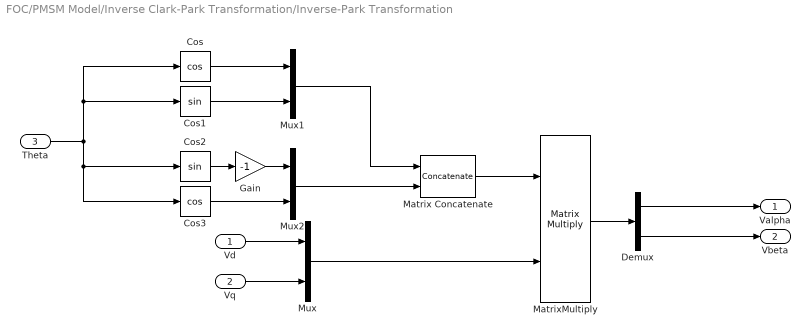
== system FOC/PMSM Model/Inverse Clark-Park Transformation/Inverse-Park Transformation ==
  Vd : Inport
  Vq : Inport  Port=2
  Theta : Inport  Port=3
  Cos : Trigonometry  Operator=cos
  Cos1 : Trigonometry
  Cos2 : Trigonometry
  Cos3 : Trigonometry  Operator=cos
  Demux : Demux  Outputs=2
  Gain : Gain  Gain=-1
  Matrix Concatenate : Concatenate  Mode=Multidimensional array  ConcatenateDimension=2
  MatrixMultiply : Product  Multiplication=Matrix(*)
  Mux : Mux  Inputs=2
  Mux1 : Mux  Inputs=2
  Mux2 : Mux  Inputs=2
  Valpha : Outport
  Vbeta : Outport  Port=2
  wires:
  Demux/2 -> Vbeta/1
  Demux/1 -> Valpha/1
  MatrixMultiply/1 -> Demux/1
  Mux/1 -> MatrixMultiply/2
  Vd/1 -> Mux/1
  Cos3/1 -> Mux2/2
  Cos1/1 -> Mux1/2
  Mux2/1 -> Matrix Concatenate/2
  Cos/1 -> Mux1/1
  Mux1/1 -> Matrix Concatenate/1
  Theta/1 -> Cos/1, Cos1/1, Cos3/1, Cos2/1
  Cos2/1 -> Gain/1
  Vq/1 -> Mux/2
  Matrix Concatenate/1 -> MatrixMultiply/1
  Gain/1 -> Mux2/1
